simulink model "asm_blocks_lib"  (R2026b)
settings: Solver=VariableStepAuto
libraries: nesl_utility x45, asmlib_lib x25, fl_lib x3, ee_lib x3
(part 2 of 3)

== system asm_blocks_lib/Messgeräte ==
  Amperemeter : Subsystem  Tag=asmlib:ammeter  mask(ASM-Bibliothek: Amperemeter){f_meas=50}
      mask prompts: f_meas "Grundfrequenz für Effektivwerte f_mess [Hz]"
      mask help:
      | Strommesser, in Reihe schalten. Positiver Strom fließt von p nach n.
      |
      | Gleichungen:
      |   I_eff = √( f_mess·∫ i² dt )  über eine Periode 1/f_mess
      |
      | Quelle: Hagl, R.: Elektrische Antriebstechnik. Hanser, München 2013
      mask Help:
      | Strommesser, in Reihe schalten. Positiver Strom fließt von p nach n.
      | 
      | Gleichungen:
      |   I_eff = √( f_mess·∫ i² dt )  über eine Periode 1/f_mess
      | 
      | Quelle: Hagl, R.: Elektrische Antriebstechnik. Hanser, München 2013
      | 
      | Parameter und Wertebereiche:
      |   f_meas         > 0, ≤ 1000  [Hz]
      | 
      | Alle Standardwerte sind Beispielwerte (parameter/asm_standard.m), keine Datenblattwerte.
      | Spezifikation: doku/SPEC.md
      mask Display:
      | plot(0.5+0.3*cos(0:0.05:6.3), 0.5+0.3*sin(0:0.05:6.3));
      | plot([0.5 0.68], [0.5 0.68]);
      | text(0.5, 0.5, 'A', 'horizontalAlignment', 'center', 'verticalAlignment', 'middle', 'texmode', 'on');
      | port_label('LConn', 1, 'p', 'texmode', 'on');
      | port_label('RConn', 1, 'n', 'texmode', 'on');
      | port_label('output', 1, 'i', 'texmode', 'on');
      | port_label('output', 2, 'I_{eff}', 'texmode', 'on');
  Drehmomentmesswelle : Subsystem  Tag=asmlib:torque_sensor  mask(ASM-Bibliothek: Drehmomentmesswelle){}
      mask help:
      | Drehmomentmesswelle, in Reihe in den Wellenstrang schalten.
      |
      | Gleichungen:
      |   M = übertragenes Wellenmoment von R nach C
      |
      | Quelle: Hagl, R.: Elektrische Antriebstechnik. Hanser, München 2013
      mask Help:
      | Drehmomentmesswelle, in Reihe in den Wellenstrang schalten.
      | 
      | Gleichungen:
      |   M = übertragenes Wellenmoment von R nach C
      | 
      | Quelle: Hagl, R.: Elektrische Antriebstechnik. Hanser, München 2013
      | 
      | Parameter und Wertebereiche:
      |   (keine)
      | 
      | Alle Standardwerte sind Beispielwerte (parameter/asm_standard.m), keine Datenblattwerte.
      | Spezifikation: doku/SPEC.md
      mask Display:
      | plot(0.5+0.3*cos(0:0.05:6.3), 0.5+0.3*sin(0:0.05:6.3));
      | plot([0.5 0.68], [0.5 0.68]);
      | text(0.5, 0.5, 'M', 'horizontalAlignment', 'center', 'verticalAlignment', 'middle', 'texmode', 'on');
      | port_label('LConn', 1, 'R', 'texmode', 'on');
      | port_label('RConn', 1, 'C', 'texmode', 'on');
      | port_label('output', 1, 'M', 'texmode', 'on');
  Drehzahlmesser : Subsystem  Tag=asmlib:speed_sensor  mask(ASM-Bibliothek: Drehzahlmesser){ns=1500}
      mask prompts: ns "Synchrondrehzahl ns (für den Schlupf) [1/min]"
      mask help:
      | Drehzahlmesser (Tacho), parallel zwischen Welle R und Bezug C.
      |
      | Gleichungen:
      |   n = 60·Ω/(2π),  s = (ns − n)/ns
      |
      | Quelle: Hagl, R.: Elektrische Antriebstechnik. Hanser, München 2013; Densborn, Skript "DS-Asynchron-Motor" (DHBW Mannheim), Folien 45-46
      mask Help:
      | Drehzahlmesser (Tacho), parallel zwischen Welle R und Bezug C.
      | 
      | Gleichungen:
      |   n = 60·Ω/(2π),  s = (ns − n)/ns
      | 
      | Quelle: Hagl, R.: Elektrische Antriebstechnik. Hanser, München 2013; Densborn, Skript "DS-Asynchron-Motor" (DHBW Mannheim), Folien 45-46
      | 
      | Parameter und Wertebereiche:
      |   ns             > 0  [1/min]
      | 
      | Alle Standardwerte sind Beispielwerte (parameter/asm_standard.m), keine Datenblattwerte.
      | Spezifikation: doku/SPEC.md
      mask Display:
      | plot(0.5+0.3*cos(0:0.05:6.3), 0.5+0.3*sin(0:0.05:6.3));
      | plot([0.5 0.68], [0.5 0.68]);
      | text(0.5, 0.5, 'n', 'horizontalAlignment', 'center', 'verticalAlignment', 'middle', 'texmode', 'on');
      | port_label('LConn', 1, 'R', 'texmode', 'on');
      | port_label('RConn', 1, 'C', 'texmode', 'on');
      | port_label('output', 1, 'n', 'texmode', 'on');
      | port_label('output', 2, 'Om', 'texmode', 'on');
      | port_label('output', 3, '\vartheta', 'texmode', 'on');
      | port_label('output', 4, 's', 'texmode', 'on');
  Leistungsmesser 3~ : Subsystem  Tag=asmlib:power_meter3  mask(ASM-Bibliothek: Leistungsmesser 3~){f_meas=50}
      mask prompts: f_meas "Grundfrequenz für Effektivwerte f_mess [Hz]"
      mask help:
      | Dreiphasiger Leistungsmesser: Strompfade in Reihe, Spannungspfade intern gegen künstlichen Sternpunkt.
      |
      | Gleichungen:
      |   p = Σ u_k·i_k,  q = [(u_b − u_c)·i_a + (u_c − u_a)·i_b + (u_a − u_b)·i_c]/√3
      |   P, Q = Mittelwerte über 1/f_mess (Q > 0 induktiv),  S = √(ΣU_k²)·√(ΣI_k²),  cos φ = P/S
      |   symmetrisch: P = √3·U·I·cos φ,  Q = √3·U·I·sin φ,  S = √3·U·I
      |
      | Quelle: Hagl, R.: Elektrische Antriebstechnik. Hanser, München 2013; Densborn, Skript "Drehstrom & Drehfeld" (DHBW Mannheim), Folie 22
      mask Help:
      | Dreiphasiger Leistungsmesser: Strompfade in Reihe, Spannungspfade intern gegen künstlichen Sternpunkt.
      | 
      | Gleichungen:
      |   p = Σ u_k·i_k,  q = [(u_b − u_c)·i_a + (u_c − u_a)·i_b + (u_a − u_b)·i_c]/√3
      |   P, Q = Mittelwerte über 1/f_mess (Q > 0 induktiv),  S = √(ΣU_k²)·√(ΣI_k²),  cos φ = P/S
      |   symmetrisch: P = √3·U·I·cos φ,  Q = √3·U·I·sin φ,  S = √3·U·I
      | 
      | Quelle: Hagl, R.: Elektrische Antriebstechnik. Hanser, München 2013; Densborn, Skript "Drehstrom & Drehfeld" (DHBW Mannheim), Folie 22
      | 
      | Parameter und Wertebereiche:
      |   f_meas         > 0, ≤ 1000  [Hz]
      | 
      | Alle Standardwerte sind Beispielwerte (parameter/asm_standard.m), keine Datenblattwerte.
      | Spezifikation: doku/SPEC.md
      mask Display:
      | plot(0.5+0.3*cos(0:0.05:6.3), 0.5+0.3*sin(0:0.05:6.3));
      | plot([0.5 0.68], [0.5 0.68]);
      | text(0.5, 0.5, 'W', 'horizontalAlignment', 'center', 'verticalAlignment', 'middle', 'texmode', 'on');
      | port_label('LConn', 1, 'a\_in', 'texmode', 'on');
      | port_label('LConn', 2, 'b\_in', 'texmode', 'on');
      | port_label('LConn', 3, 'c\_in', 'texmode', 'on');
      | port_label('RConn', 1, 'a\_out', 'texmode', 'on');
      | port_label('RConn', 2, 'b\_out', 'texmode', 'on');
      | port_label('RConn', 3, 'c\_out', 'texmode', 'on');
      | port_label('output', 1, 'P', 'texmode', 'on');
      | port_label('output', 2, 'Q', 'texmode', 'on');
      | port_label('output', 3, 'S', 'texmode', 'on');
      | port_label('output', 4, 'cosphi', 'texmode', 'on');
  Luftspalt-Sonde : Subsystem  Tag=asmlib:airgap_probe  mask(ASM-Bibliothek: Luftspalt-Sonde){p=2, N1xi1=144, l=0.15, r=0.06}
      mask prompts: p "Polpaarzahl p [-]"; N1xi1 "wirksame Windungszahl N1·ξ1 [-]"; l "wirksame Stablänge l [m]"; r "Radius der Stabmitte r [m]"
      mask help:
      | Misst das Drehfeld im Luftspalt (wie eine Hallsonde), parallel am Port LS anschließen.
      |
      | Gleichungen:
      |   ψh = Across-Größe am Port LS
      |   φ_el = ∠ψh,   B̂ = p·|ψh| / (2·N1ξ1·l·r),   B(γ,t) = B̂·cos(γ − φ_el)
      |
      | Quelle: Hagl, R.: Elektrische Antriebstechnik. Hanser, München 2013; Densborn, Skript "DS-Asynchron-Motor" (DHBW Mannheim), Folie 14
      mask Help:
      | Misst das Drehfeld im Luftspalt (wie eine Hallsonde), parallel am Port LS anschließen.
      | 
      | Gleichungen:
      |   ψh = Across-Größe am Port LS
      |   φ_el = ∠ψh,   B̂ = p·|ψh| / (2·N1ξ1·l·r),   B(γ,t) = B̂·cos(γ − φ_el)
      | 
      | Quelle: Hagl, R.: Elektrische Antriebstechnik. Hanser, München 2013; Densborn, Skript "DS-Asynchron-Motor" (DHBW Mannheim), Folie 14
      | 
      | Parameter und Wertebereiche:
      |   p              ganzzahlig, ≥ 1, ≤ 12  [-]
      |   N1xi1          > 0  [-]
      |   l              > 0  [m]
      |   r              > 0  [m]
      | 
      | Alle Standardwerte sind Beispielwerte (parameter/asm_standard.m), keine Datenblattwerte.
      | Spezifikation: doku/SPEC.md
      mask Display:
      | plot(0.5+0.3*cos(0:0.05:6.3), 0.5+0.3*sin(0:0.05:6.3));
      | plot([0.5 0.68], [0.5 0.68]);
      | text(0.5, 0.5, 'B', 'horizontalAlignment', 'center', 'verticalAlignment', 'middle', 'texmode', 'on');
      | port_label('LConn', 1, 'LS', 'texmode', 'on');
      | port_label('output', 1, '\psi_h', 'texmode', 'on');
      | port_label('output', 2, '\phi_{el}', 'texmode', 'on');
      | port_label('output', 3, 'Bhat', 'texmode', 'on');
  Schreiber : Subsystem  Tag=asmlib:recorder  mask(ASM-Bibliothek: Schreiber){title_text=Messung}
      mask prompts: title_text "Titel (erscheint auf dem Baustein)"
      mask help:
      | Messschreiber (Simulink Scope). Mehrere Signale über einen Mux anschließen; das Scope zeigt
      | die Signalnamen. Für Folienbilder die Signale protokollieren und mit asmexport.slide_figure exportieren.
      |
      | Gleichungen:
      |   –
      |
      | Quelle: Hagl, R.: Elektrische Antriebstechnik. Hanser, München 2013
      mask Help:
      | Messschreiber (Simulink Scope). Mehrere Signale über einen Mux anschließen; das Scope zeigt
      | die Signalnamen. Für Folienbilder die Signale protokollieren und mit asmexport.slide_figure exportieren.
      | 
      | Gleichungen:
      |   –
      | 
      | Quelle: Hagl, R.: Elektrische Antriebstechnik. Hanser, München 2013
      | 
      | Parameter und Wertebereiche:
      |   title_text     Text
      | 
      | Alle Standardwerte sind Beispielwerte (parameter/asm_standard.m), keine Datenblattwerte.
      | Spezifikation: doku/SPEC.md
      mask Display:
      | plot(0.5+0.3*cos(0:0.05:6.3), 0.5+0.3*sin(0:0.05:6.3));
      | plot([0.5 0.68], [0.5 0.68]);
      | text(0.5, 0.6, 'Schreiber', 'horizontalAlignment', 'center');
      | text(0.5, 0.3, title_text, 'horizontalAlignment', 'center');
      | port_label('input', 1, 'u', 'texmode', 'on');
  Spannungsmessung 3~ : Subsystem  Tag=asmlib:voltage_sensor3  mask(ASM-Bibliothek: Spannungsmessung 3~){f_meas=50, reference=künstlicher Sternpunkt}
      mask prompts: f_meas "Grundfrequenz für Effektivwerte f_mess [Hz]"; reference "Bezug der Strangspannungen"
      mask help:
      | Dreiphasige Spannungsmessung, parallel anschließen. Strangspannungen gegen den künstlichen
      | Sternpunkt oder gegen den Anschluss n (dann muss n angeschlossen sein). U_eff = Leiterspannung.
      |
      | Gleichungen:
      |   u_Str,k = v_k − v_m,  v_m = (v_a + v_b + v_c)/3 bzw. v_n;  u_ab = v_a − v_b, …
      |   U_eff = √(f_mess/3·∫(u_ab² + u_bc² + u_ca²) dt);  symmetrisch U = √3·U_Str
      |
      | Quelle: Hagl, R.: Elektrische Antriebstechnik. Hanser, München 2013; Densborn, Skript "Drehstrom & Drehfeld" (DHBW Mannheim), Folien 11-16
      mask Help:
      | Dreiphasige Spannungsmessung, parallel anschließen. Strangspannungen gegen den künstlichen
      | Sternpunkt oder gegen den Anschluss n (dann muss n angeschlossen sein). U_eff = Leiterspannung.
      | 
      | Gleichungen:
      |   u_Str,k = v_k − v_m,  v_m = (v_a + v_b + v_c)/3 bzw. v_n;  u_ab = v_a − v_b, …
      |   U_eff = √(f_mess/3·∫(u_ab² + u_bc² + u_ca²) dt);  symmetrisch U = √3·U_Str
      | 
      | Quelle: Hagl, R.: Elektrische Antriebstechnik. Hanser, München 2013; Densborn, Skript "Drehstrom & Drehfeld" (DHBW Mannheim), Folien 11-16
      | 
      | Parameter und Wertebereiche:
      |   f_meas         > 0, ≤ 1000  [Hz]
      |   reference      Auswahl: künstlicher Sternpunkt | Anschluss n
      | 
      | Alle Standardwerte sind Beispielwerte (parameter/asm_standard.m), keine Datenblattwerte.
      | Spezifikation: doku/SPEC.md
      mask TypeOptions reference: künstlicher Sternpunkt | Anschluss n
      mask Display:
      | plot(0.5+0.3*cos(0:0.05:6.3), 0.5+0.3*sin(0:0.05:6.3));
      | plot([0.5 0.68], [0.5 0.68]);
      | text(0.5, 0.5, 'V 3~', 'horizontalAlignment', 'center', 'verticalAlignment', 'middle', 'texmode', 'on');
      | port_label('LConn', 1, 'a', 'texmode', 'on');
      | port_label('LConn', 2, 'b', 'texmode', 'on');
      | port_label('LConn', 3, 'c', 'texmode', 'on');
      | port_label('LConn', 4, 'n', 'texmode', 'on');
      | port_label('output', 1, 'u_{phase}', 'texmode', 'on');
      | port_label('output', 2, 'u_{line}', 'texmode', 'on');
      | port_label('output', 3, 'U_{eff}', 'texmode', 'on');
  Strommessung 3~ : Subsystem  Tag=asmlib:current_sensor3  mask(ASM-Bibliothek: Strommessung 3~){f_meas=50}
      mask prompts: f_meas "Grundfrequenz für Effektivwerte f_mess [Hz]"
      mask help:
      | Dreiphasige Strommessung, in Reihe in die drei Leiter schalten.
      |
      | Gleichungen:
      |   i1 = 2/3·(i_a + a·i_b + a²·i_c)  (Raumzeiger)
      |   I_eff = √(f_mess/3·∫(i_a² + i_b² + i_c²) dt)  (quadratischer Mittelwert der drei Leiter)
      |
      | Quelle: Hagl, R.: Elektrische Antriebstechnik. Hanser, München 2013; Densborn, Skript "Drehstrom & Drehfeld" (DHBW Mannheim)
      mask Help:
      | Dreiphasige Strommessung, in Reihe in die drei Leiter schalten.
      | 
      | Gleichungen:
      |   i1 = 2/3·(i_a + a·i_b + a²·i_c)  (Raumzeiger)
      |   I_eff = √(f_mess/3·∫(i_a² + i_b² + i_c²) dt)  (quadratischer Mittelwert der drei Leiter)
      | 
      | Quelle: Hagl, R.: Elektrische Antriebstechnik. Hanser, München 2013; Densborn, Skript "Drehstrom & Drehfeld" (DHBW Mannheim)
      | 
      | Parameter und Wertebereiche:
      |   f_meas         > 0, ≤ 1000  [Hz]
      | 
      | Alle Standardwerte sind Beispielwerte (parameter/asm_standard.m), keine Datenblattwerte.
      | Spezifikation: doku/SPEC.md
      mask Display:
      | plot(0.5+0.3*cos(0:0.05:6.3), 0.5+0.3*sin(0:0.05:6.3));
      | plot([0.5 0.68], [0.5 0.68]);
      | text(0.5, 0.5, 'A 3~', 'horizontalAlignment', 'center', 'verticalAlignment', 'middle', 'texmode', 'on');
      | port_label('LConn', 1, 'a\_in', 'texmode', 'on');
      | port_label('LConn', 2, 'b\_in', 'texmode', 'on');
      | port_label('LConn', 3, 'c\_in', 'texmode', 'on');
      | port_label('RConn', 1, 'a\_out', 'texmode', 'on');
      | port_label('RConn', 2, 'b\_out', 'texmode', 'on');
      | port_label('RConn', 3, 'c\_out', 'texmode', 'on');
      | port_label('output', 1, 'i_{abc}', 'texmode', 'on');
      | port_label('output', 2, 'I_{eff}', 'texmode', 'on');
      | port_label('output', 3, 'i1', 'texmode', 'on');
  Voltmeter : Subsystem  Tag=asmlib:voltmeter  mask(ASM-Bibliothek: Voltmeter){f_meas=50}
      mask prompts: f_meas "Grundfrequenz für Effektivwerte f_mess [Hz]"
      mask help:
      | Spannungsmesser, parallel schalten. u = v_p − v_n.
      |
      | Gleichungen:
      |   U_eff = √( f_mess·∫ u² dt )  über eine Periode 1/f_mess
      |
      | Quelle: Hagl, R.: Elektrische Antriebstechnik. Hanser, München 2013
      mask Help:
      | Spannungsmesser, parallel schalten. u = v_p − v_n.
      | 
      | Gleichungen:
      |   U_eff = √( f_mess·∫ u² dt )  über eine Periode 1/f_mess
      | 
      | Quelle: Hagl, R.: Elektrische Antriebstechnik. Hanser, München 2013
      | 
      | Parameter und Wertebereiche:
      |   f_meas         > 0, ≤ 1000  [Hz]
      | 
      | Alle Standardwerte sind Beispielwerte (parameter/asm_standard.m), keine Datenblattwerte.
      | Spezifikation: doku/SPEC.md
      mask Display:
      | plot(0.5+0.3*cos(0:0.05:6.3), 0.5+0.3*sin(0:0.05:6.3));
      | plot([0.5 0.68], [0.5 0.68]);
      | text(0.5, 0.5, 'V', 'horizontalAlignment', 'center', 'verticalAlignment', 'middle', 'texmode', 'on');
      | port_label('LConn', 1, 'p', 'texmode', 'on');
      | port_label('RConn', 1, 'n', 'texmode', 'on');
      | port_label('output', 1, 'u', 'texmode', 'on');
      | port_label('output', 2, 'U_{eff}', 'texmode', 'on');

== system asm_blocks_lib/Quellen ==
  Netz 3~ : Subsystem  Tag=asmlib:grid3  mask(ASM-Bibliothek: Netz 3~){U_L=400, f1=50, phase_seq=L1-L2-L3 (Rechtsdrehfeld), phi0=0, t_on=0, R_N=0, L_N=0}
      mask prompts: U_L "Leiterspannung U (Effektivwert) [V]"; f1 "Frequenz f1 [Hz]"; phase_seq "Phasenfolge"; phi0 "Nullphasenwinkel von L1 [°]"; t_on "Einschaltzeitpunkt t_ein [s]"; R_N "Netzinnenwiderstand je Leiter R_N [Ω]"; L_N "Netzinneninduktivität je Leiter L_N [H]"
      mask help:
      | Symmetrisches Drehstromnetz, Sternpunkt n herausgeführt, optional mit Innenimpedanz (R_N = L_N = 0: starres Netz).
      |
      | Gleichungen:
      |   u_L1 = √2·U/√3·sin(ω1·t + φ0),  u_L2 = √2·U/√3·sin(ω1·t + φ0 − 2π/3),
      |   u_L3 = √2·U/√3·sin(ω1·t + φ0 − 4π/3)  (Rechtsdrehfeld),  ω1 = 2π·f1
      |   Spannung liegt ab t ≥ t_ein an.
      |
      | Quelle: Hagl, R.: Elektrische Antriebstechnik. Hanser, München 2013; Densborn, Skript "Drehstrom & Drehfeld" (DHBW Mannheim), Folien 8-12
      mask Help:
      | Symmetrisches Drehstromnetz, Sternpunkt n herausgeführt, optional mit Innenimpedanz (R_N = L_N = 0: starres Netz).
      | 
      | Gleichungen:
      |   u_L1 = √2·U/√3·sin(ω1·t + φ0),  u_L2 = √2·U/√3·sin(ω1·t + φ0 − 2π/3),
      |   u_L3 = √2·U/√3·sin(ω1·t + φ0 − 4π/3)  (Rechtsdrehfeld),  ω1 = 2π·f1
      |   Spannung liegt ab t ≥ t_ein an.
      | 
      | Quelle: Hagl, R.: Elektrische Antriebstechnik. Hanser, München 2013; Densborn, Skript "Drehstrom & Drehfeld" (DHBW Mannheim), Folien 8-12
      | 
      | Parameter und Wertebereiche:
      |   U_L            ≥ 0, ≤ 1e4  [V]
      |   f1             > 0, ≤ 1000  [Hz]
      |   phase_seq      Auswahl: L1-L2-L3 (Rechtsdrehfeld) | L1-L3-L2 (Linksdrehfeld)
      |   phi0           ≥ -360, ≤ 360  [°]
      |   t_on           ≥ 0  [s]
      |   R_N            ≥ 0  [Ω]
      |   L_N            ≥ 0  [H]
      | 
      | Alle Standardwerte sind Beispielwerte (parameter/asm_standard.m), keine Datenblattwerte.
      | Spezifikation: doku/SPEC.md
      mask TypeOptions phase_seq: L1-L2-L3 (Rechtsdrehfeld) | L1-L3-L2 (Linksdrehfeld)
      mask Display:
      | plot(0.5+0.3*cos(0:0.05:6.3), 0.5+0.3*sin(0:0.05:6.3));
      | text(0.5, 0.5, '3~', 'horizontalAlignment', 'center', 'verticalAlignment', 'middle', 'texmode', 'on');
      | port_label('RConn', 1, 'a', 'texmode', 'on');
      | port_label('RConn', 2, 'b', 'texmode', 'on');
      | port_label('RConn', 3, 'c', 'texmode', 'on');
      | port_label('RConn', 4, 'n', 'texmode', 'on');
  Sternpunkt (Erde) : Subsystem  Tag=asmlib:neutral_ground  mask(ASM-Bibliothek: Sternpunkt (Erde)){}
      mask help:
      | Elektrisches Bezugspotenzial (0 V). Jedes elektrische Netzwerk braucht mindestens einen Bezug.
      |
      | Gleichungen:
      |   u_N = 0
      |
      | Quelle: Hagl, R.: Elektrische Antriebstechnik. Hanser, München 2013
      mask Help:
      | Elektrisches Bezugspotenzial (0 V). Jedes elektrische Netzwerk braucht mindestens einen Bezug.
      | 
      | Gleichungen:
      |   u_N = 0
      | 
      | Quelle: Hagl, R.: Elektrische Antriebstechnik. Hanser, München 2013
      | 
      | Parameter und Wertebereiche:
      |   (keine)
      | 
      | Alle Standardwerte sind Beispielwerte (parameter/asm_standard.m), keine Datenblattwerte.
      | Spezifikation: doku/SPEC.md
      mask Display:
      | plot(0.5+0.3*cos(0:0.05:6.3), 0.5+0.3*sin(0:0.05:6.3));
      | text(0.5, 0.5, '\perp', 'horizontalAlignment', 'center', 'verticalAlignment', 'middle', 'texmode', 'on');
      | port_label('LConn', 1, 'N', 'texmode', 'on');

== system asm_blocks_lib/Referenz ==
  ASM Kloss (quasistationär) : Subsystem  Tag=asmlib:asm_kloss  mask(ASM-Bibliothek: ASM Kloss (quasistationär)){MK=71.55, sK=0.2, ns=1500}
      mask prompts: MK "Kippmoment MK [N·m]"; sK "Kippschlupf sK [-]"; ns "Synchrondrehzahl ns [1/min]"
      mask help:
      | Quasistationäres Motormoment nach Kloss (Teil B des Prototyps, R1 = 0, konstanter Fluss,
      | keine elektrische Dynamik, keine eigene Trägheit: J_M als Schwungmasse anschließen).
      |
      | Gleichungen:
      |   M = 2·MK·s·sK / (s² + sK²),   s = (ns − n)/ns
      |
      | Quelle: Hagl, R.: Elektrische Antriebstechnik. Hanser, München 2013; Densborn, Skript "DS-Asynchron-Motor" (DHBW Mannheim), Folien 47-50
      mask Help:
      | Quasistationäres Motormoment nach Kloss (Teil B des Prototyps, R1 = 0, konstanter Fluss,
      | keine elektrische Dynamik, keine eigene Trägheit: J_M als Schwungmasse anschließen).
      | 
      | Gleichungen:
      |   M = 2·MK·s·sK / (s² + sK²),   s = (ns − n)/ns
      | 
      | Quelle: Hagl, R.: Elektrische Antriebstechnik. Hanser, München 2013; Densborn, Skript "DS-Asynchron-Motor" (DHBW Mannheim), Folien 47-50
      | 
      | Parameter und Wertebereiche:
      |   MK             > 0  [N·m]
      |   sK             > 0, ≤ 1  [-]
      |   ns             > 0  [1/min]
      | 
      | Alle Standardwerte sind Beispielwerte (parameter/asm_standard.m), keine Datenblattwerte.
      | Spezifikation: doku/SPEC.md
      mask Display:
      | plot([0.1 0.9], [0.1 0.1]); plot([0.1 0.9], [0.9 0.9]);
      | text(0.5, 0.5, 'Kloss', 'horizontalAlignment', 'center', 'verticalAlignment', 'middle', 'texmode', 'on');
      | port_label('RConn', 1, 'R', 'texmode', 'on');
      | port_label('RConn', 2, 'C', 'texmode', 'on');
      | port_label('output', 1, 'M', 'texmode', 'on');
      | port_label('output', 2, 's', 'texmode', 'on');
  ASM Referenz (Simscape Electrical) : Subsystem  Tag=asmlib:asm_reference  mask(ASM-Bibliothek: ASM Referenz (Simscape Electrical)){param_set=Standard, U_N=400, f_N=50, p=2, R1=0.5, L1s=0.009902, Lh=0.25, R2b=1.225, L2sb=0.009902, J_M=0.012}
      mask prompts: param_set "Parametersatz"; U_N "Bemessungsspannung U_N (Leiter, eff.) [V]"; f_N "Bemessungsfrequenz f_N [Hz]"; p "Polpaarzahl p [-]"; R1 "Statorwiderstand R1 [Ω]"; L1s "Statorstreuinduktivität L1σ [H]"; Lh "Hauptinduktivität Lh [H]"; R2b "Rotorwiderstand R2′ (statorbezogen) [Ω]"; L2sb "Rotorstreuinduktivität L2σ′ (statorbezogen) [H]"; J_M "Trägheitsmoment Motor J_M [kg·m²]"
      mask help:
      | Referenzmotor mit "Induction Machine Squirrel Cage" aus Simscape Electrical (ee_lib) und demselben
      | Parametersatz wie "ASM Standard" (Sternschaltung, Sternpunkt frei, Start stromlos). J_M liegt als
      | Schwungmasse an der Welle R. Nur zum Modellvergleich (Benchmark), keine Messung.
      | Hinweis: Die ee_lib-Maschine verträgt keine Solver-Ereignisse (Sprünge, unstetige Funktionen)
      | im selben Modell; alle Bausteine der Bibliothek sind deshalb ereignisfrei formuliert.
      |
      | Gleichungen:
      | Raumzeigermodell, statorfest (Index 1 = Stator, 2 = Rotor, ′ = statorbezogen):
      |   u1 = R1·i1 + dψ1/dt
      |   0  = R2′·i2′ + dψ2′/dt − j·p·Ω·ψ2′
      |   ψ1 = L1σ·i1 + ψh,   ψ2′ = L2σ′·i2′ + ψh,   ψh = Lh·(i1 + i2′)
      |   M  = 3/2·p·Im{ψh*·i1},   J·dΩ/dt = M − M_L − k_R·Ω
      |   n = 60·Ω/(2π),   s = (ns − n)/ns,   ns = 60·f1/p
      |
      | Quelle: Hagl, R.: Elektrische Antriebstechnik. Hanser, München 2013
      mask init:
      | % parameter set "Standard": values from parameter/asm_standard.m
      | if param_set == 1
      |     S = asm_standard();
      |     U_N = S.U_N; f_N = S.f_N; p = S.p; R1 = S.R1; L1s = S.L1s; Lh = S.Lh; R2b = S.R2b; L2sb = S.L2sb; J_M = S.J_M;
      | end
      mask Help:
      | Referenzmotor mit "Induction Machine Squirrel Cage" aus Simscape Electrical (ee_lib) und demselben
      | Parametersatz wie "ASM Standard" (Sternschaltung, Sternpunkt frei, Start stromlos). J_M liegt als
      | Schwungmasse an der Welle R. Nur zum Modellvergleich (Benchmark), keine Messung.
      | Hinweis: Die ee_lib-Maschine verträgt keine Solver-Ereignisse (Sprünge, unstetige Funktionen)
      | im selben Modell; alle Bausteine der Bibliothek sind deshalb ereignisfrei formuliert.
      | 
      | Gleichungen:
      | Raumzeigermodell, statorfest (Index 1 = Stator, 2 = Rotor, ′ = statorbezogen):
      |   u1 = R1·i1 + dψ1/dt
      |   0  = R2′·i2′ + dψ2′/dt − j·p·Ω·ψ2′
      |   ψ1 = L1σ·i1 + ψh,   ψ2′ = L2σ′·i2′ + ψh,   ψh = Lh·(i1 + i2′)
      |   M  = 3/2·p·Im{ψh*·i1},   J·dΩ/dt = M − M_L − k_R·Ω
      |   n = 60·Ω/(2π),   s = (ns − n)/ns,   ns = 60·f1/p
      | 
      | Quelle: Hagl, R.: Elektrische Antriebstechnik. Hanser, München 2013
      | 
      | Parameter und Wertebereiche:
      |   param_set      Auswahl: Standard | Benutzerdefiniert
      |   U_N            > 0, ≤ 1e4  [V]
      |   f_N            > 0, ≤ 1000  [Hz]
      |   p              ganzzahlig, ≥ 1, ≤ 12  [-]
      |   R1             > 0  [Ω]
      |   L1s            > 0  [H]
      |   Lh             > 0  [H]
      |   R2b            > 0  [Ω]
      |   L2sb           > 0  [H]
      |   J_M            > 0  [kg·m²]
      | 
      | Alle Standardwerte sind Beispielwerte (parameter/asm_standard.m), keine Datenblattwerte.
      | Spezifikation: doku/SPEC.md
      mask TypeOptions param_set: Standard | Benutzerdefiniert
      mask Callback param_set: asmtools.param_set_callback(gcb);
      mask Display:
      | plot([0.1 0.9], [0.1 0.1]); plot([0.1 0.9], [0.9 0.9]);
      | text(0.5, 0.5, 'Referenz', 'horizontalAlignment', 'center', 'verticalAlignment', 'middle', 'texmode', 'on');
      | port_label('LConn', 1, 'a', 'texmode', 'on');
      | port_label('LConn', 2, 'b', 'texmode', 'on');
      | port_label('LConn', 3, 'c', 'texmode', 'on');
      | port_label('RConn', 1, 'R', 'texmode', 'on');
      | port_label('RConn', 2, 'C', 'texmode', 'on');
  Leiterschleife (Prototyp Teil A) : Subsystem  Tag=asmlib:conductor_loop  mask(ASM-Bibliothek: Leiterschleife (Prototyp Teil A)){Bhat=0.8, l=0.15, r=0.06, f1=50, p=2, R2_S=0.000318664, L2s_S=5.0717e-06, conv_phi2=+1, phi2_mode=aus Rotorimpedanz, phi2_fix=90}
      mask prompts: Bhat "Amplitude der Luftspaltflussdichte B̂ [T]"; l "wirksame Stablänge l [m]"; r "Radius der Stabmitte r [m]"; f1 "Statorfrequenz f1 [Hz]"; p "Polpaarzahl p [-]"; R2_S "Widerstand der Leiterschleife R2 [Ω]"; L2s_S "Streuinduktivität der Leiterschleife L2σ [H]"; conv_phi2 "Vorzeichenkonvention konv_phi2"; phi2_mode "Versatzwinkel φ2"; phi2_fix "fester Versatzwinkel φ2 [°]"
      mask help:
      | Leiterschleife aus zwei Rotorstäben im rotorfesten System (Teil A des Prototyps), Eingang Schlupf s.
      | Der Schlupf ist eine Vorgabe (Konstante oder Signal); das Schleifenmoment wirkt nicht auf die Mechanik
      | zurück. R2 und L2σ sind aus MK und sK abgeleitet (parameter/asm_standard.m).
      |
      | Gleichungen:
      |   θ2 = ∫ s·ω1 dt,  B_k = B̂·cos(γ_k − θ2),  i_k = î2·sin(γ_k − θ2 + konv·φ2)
      |   F_k = konv·i_k·l·B_k,  M_k = F_k·r,  M_S = M_1 + M_2
      |
      | Quelle: Hagl, R.: Elektrische Antriebstechnik. Hanser, München 2013; Densborn, Skript "DS-Asynchron-Motor" (DHBW Mannheim), Folien 14-16
      mask Help:
      | Leiterschleife aus zwei Rotorstäben im rotorfesten System (Teil A des Prototyps), Eingang Schlupf s.
      | Der Schlupf ist eine Vorgabe (Konstante oder Signal); das Schleifenmoment wirkt nicht auf die Mechanik
      | zurück. R2 und L2σ sind aus MK und sK abgeleitet (parameter/asm_standard.m).
      | 
      | Gleichungen:
      |   θ2 = ∫ s·ω1 dt,  B_k = B̂·cos(γ_k − θ2),  i_k = î2·sin(γ_k − θ2 + konv·φ2)
      |   F_k = konv·i_k·l·B_k,  M_k = F_k·r,  M_S = M_1 + M_2
      | 
      | Quelle: Hagl, R.: Elektrische Antriebstechnik. Hanser, München 2013; Densborn, Skript "DS-Asynchron-Motor" (DHBW Mannheim), Folien 14-16
      | 
      | Parameter und Wertebereiche:
      |   Bhat           > 0, ≤ 2.5  [T]
      |   l              > 0  [m]
      |   r              > 0  [m]
      |   f1             > 0, ≤ 1000  [Hz]
      |   p              ganzzahlig, ≥ 1, ≤ 12  [-]
      |   R2_S           > 0  [Ω]
      |   L2s_S          > 0  [H]
      |   conv_phi2      Auswahl: +1 | -1
      |   phi2_mode      Auswahl: aus Rotorimpedanz | fest
      |   phi2_fix       ≥ 0, ≤ 180  [°]
      | 
      | Alle Standardwerte sind Beispielwerte (parameter/asm_standard.m), keine Datenblattwerte.
      | Spezifikation: doku/SPEC.md
      mask TypeOptions conv_phi2: +1 | -1
      mask TypeOptions phi2_mode: aus Rotorimpedanz | fest
      mask Display:
      | plot([0.1 0.9], [0.1 0.1]); plot([0.1 0.9], [0.9 0.9]);
      | text(0.5, 0.5, 'Schleife', 'horizontalAlignment', 'center', 'verticalAlignment', 'middle', 'texmode', 'on');
      | port_label('input', 1, 's', 'texmode', 'on');
      | port_label('output', 1, 'B_k', 'texmode', 'on');
      | port_label('output', 2, 'i_k', 'texmode', 'on');
      | port_label('output', 3, 'F_k', 'texmode', 'on');
      | port_label('output', 4, 'M_k', 'texmode', 'on');
      | port_label('output', 5, 'M_S', 'texmode', 'on');
      | port_label('output', 6, 'B_\perp', 'texmode', 'on');
      | port_label('output', 7, '\phi2', 'texmode', 'on');
      | port_label('output', 8, 'i2hat', 'texmode', 'on');
      | port_label('output', 9, '\theta_2', 'texmode', 'on');

== system asm_blocks_lib/Didaktik/Drehfeld-Anzeige ==
  psi_h : Inport
  i2b : Inport  Port=2
  th_mech : Inport  Port=3
  Log : ToWorkspace  VariableName=field_display_log  SaveFormat=Structure With Time  SampleTime=-1
  Mux : Mux  Inputs=[2 2 1]
  wires:
  psi_h/1 -> Mux/1
  i2b/1 -> Mux/2
  th_mech/1 -> Mux/3
  Mux/1 -> Log/1

== system asm_blocks_lib/Didaktik/Ideales Drehfeld ==
  Clock : Clock
  Field : MATLABSystem  System=asmtools.IdealRotatingField  Bhat=Bhat  f1=f1  p=p  s=s  l=l  r=r  N1xi1=N1xi1  N2=N2  R2_S=R2_S  L2s_S=L2s_S  mode=phi2_mode  phi2_fix=phi2_fix  SimulateUsing=Interpreted execution
      mask Type: asmtools.IdealRotatingField
  psi_h : Outport
  i2b : Outport  Port=2
  th_mech : Outport  Port=3
  phi_el : Outport  Port=4
  phi2 : Outport  Port=5
  wires:
  Clock/1 -> Field/1
  Field/1 -> psi_h/1
  Field/2 -> i2b/1
  Field/3 -> th_mech/1
  Field/4 -> phi_el/1
  Field/5 -> phi2/1

== system asm_blocks_lib/Didaktik/Kennlinienschreiber ==
  n : Inport
  M : Inport  Port=2
  M_L : Inport  Port=3
  Log : ToWorkspace  VariableName=torque_speed_log  SaveFormat=Structure With Time  SampleTime=-1
  Mux : Mux  Inputs=3
  wires:
  n/1 -> Mux/1
  M/1 -> Mux/2
  M_L/1 -> Mux/3
  Mux/1 -> Log/1

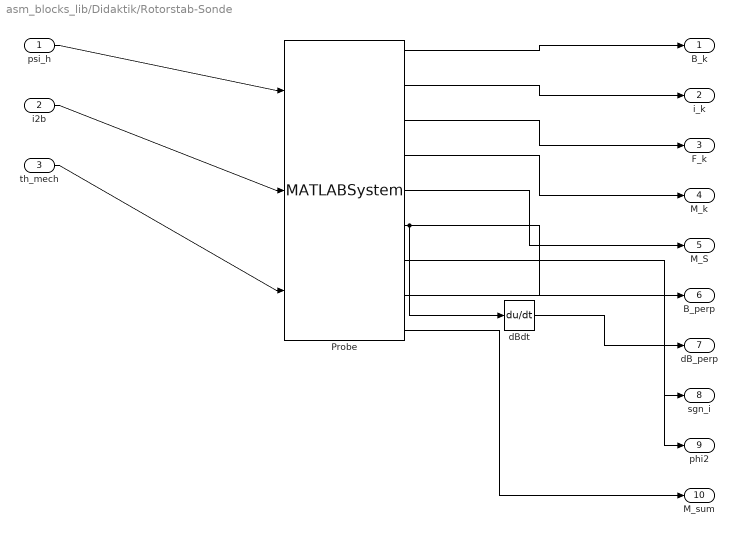
== system asm_blocks_lib/Didaktik/Rotorstab-Sonde ==
  psi_h : Inport
  i2b : Inport  Port=2
  th_mech : Inport  Port=3
  Probe : MATLABSystem  System=asmtools.RotorBarProbe  p=p  N2=N2  l=l  r=r  N1xi1=N1xi1  k1=k1  k2=k2  bar1_angle=bar1_angle*pi/180  slide_convention=convention == 1  SimulateUsing=Interpreted execution
      mask Type: asmtools.RotorBarProbe
  dBdt : Derivative
  B_k : Outport
  i_k : Outport  Port=2
  F_k : Outport  Port=3
  M_k : Outport  Port=4
  M_S : Outport  Port=5
  B_perp : Outport  Port=6
  dB_perp : Outport  Port=7
  sgn_i : Outport  Port=8
  phi2 : Outport  Port=9
  M_sum : Outport  Port=10
  wires:
  psi_h/1 -> Probe/1
  i2b/1 -> Probe/2
  th_mech/1 -> Probe/3
  Probe/6 -> dBdt/1, B_perp/1
  Probe/1 -> B_k/1
  Probe/2 -> i_k/1
  Probe/3 -> F_k/1
  Probe/4 -> M_k/1
  Probe/5 -> M_S/1
  dBdt/1 -> dB_perp/1
  Probe/7 -> sgn_i/1
  Probe/8 -> phi2/1
  Probe/9 -> M_sum/1

== system asm_blocks_lib/Didaktik/Spulenfelder ==
  i_abc : Inport
  f_BUVW : Gain  Gain=p*Lh/(2*N1xi1*l*r)*2/3
  f_Bhat : Fcn  Expr=p*Lh/(2*N1xi1*l*r)*sqrt((2/3*(u(1)-u(2)/2-u(3)/2))^2 + ((u(2)-u(3))/sqrt(3))^2)
  f_phi : Fcn  Expr=atan2((u(2)-u(3))/sqrt(3), 2/3*(u(1)-u(2)/2-u(3)/2))
  B_UVW : Outport
  Bhat : Outport  Port=2
  phi_el : Outport  Port=3
  wires:
  i_abc/1 -> f_BUVW/1, f_Bhat/1, f_phi/1
  f_BUVW/1 -> B_UVW/1
  f_Bhat/1 -> Bhat/1
  f_phi/1 -> phi_el/1

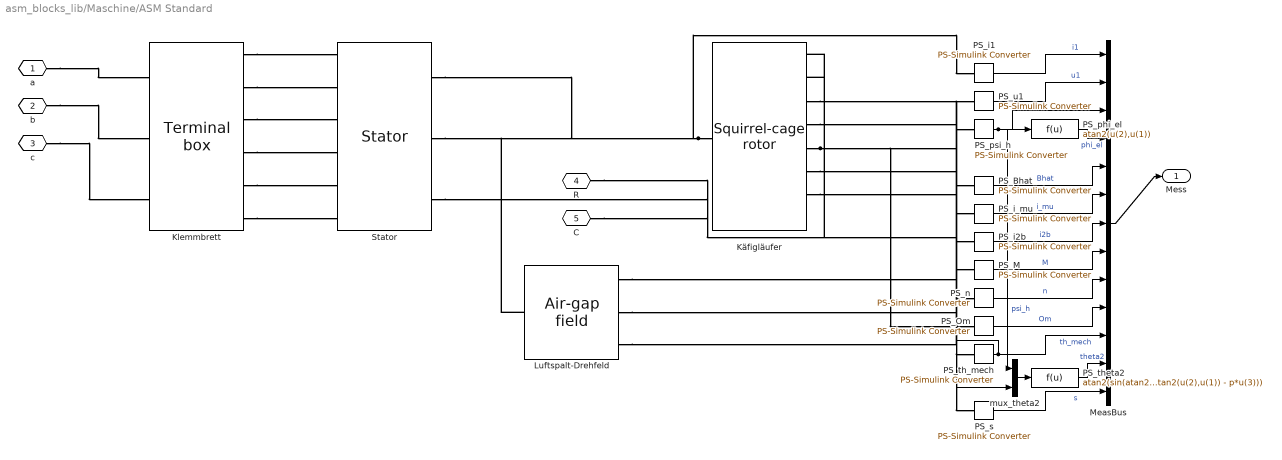
== system asm_blocks_lib/Maschine/ASM Standard ==
  Klemmbrett : asmlib_lib/machine/Terminal box  connection=connection  i_aU1_specify=off  i_aU1_priority=None  i_aU1=0 A  i_aU1_nominal_specify=off  i_aU1_nominal_value=1  i_aU1_nominal_unit=A  i_bV1_specify=off  i_bV1_priority=None  i_bV1=0 A  i_bV1_nominal_specify=off  i_bV1_nominal_value=1  i_bV1_nominal_unit=A  i_cW1_specify=off  i_cW1_priority=None  i_cW1=0 A  i_cW1_nominal_specify=off  i_cW1_nominal_value=1  i_cW1_nominal_unit=A  i_aW2_specify=off  i_aW2_priority=None  i_aW2=0 A  i_aW2_nominal_specify=off  i_aW2_nominal_value=1  i_aW2_nominal_unit=A  i_bU2_specify=off  i_bU2_priority=None  i_bU2=0 A  i_bU2_nominal_specify=off  i_bU2_nominal_value=1  i_bU2_nominal_unit=A  i_cV2_specify=off  i_cV2_priority=None  i_cV2=0 A  i_cV2_nominal_specify=off  i_cV2_nominal_value=1  i_cV2_nominal_unit=A  i_UV2_specify=off  i_UV2_priority=None  i_UV2=0 A  i_UV2_nominal_specify=off  i_UV2_nominal_value=1  i_UV2_nominal_unit=A  i_VW2_specify=off  i_VW2_priority=None  i_VW2=0 A  i_VW2_nominal_specify=off  i_VW2_nominal_value=1  i_VW2_nominal_unit=A
  Käfigläufer : asmlib_lib/machine/Squirrel-cage rotor  R2b=R2b Ohm  L2sb=L2sb H  p=p  f_N=f_N Hz  J_M=J_M kg*m^2  k_R=k_R N*m*s/rad  n0=n0 rpm  i2_specify=off  i2_priority=None  i2=zeros(2, 1) A  i2_nominal_specify=off  i2_nominal_value=1  i2_nominal_unit=A  psih_specify=off  psih_priority=None  psih=zeros(2, 1) Wb  psih_nominal_specify=off  psih_nominal_value=1  psih_nominal_unit=Wb  psi2_specify=off  psi2_priority=None  psi2=zeros(2, 1) Wb  psi2_nominal_specify=off  psi2_nominal_value=1  psi2_nominal_unit=Wb  psi2r_specify=off  psi2r_priority=High  psi2r=zeros(2, 1) Wb  psi2r_nominal_specify=off  psi2r_nominal_value=1  psi2r_nominal_unit=Wb  th_specify=off  th_priority=High  th=0 rad  th_nominal_specify=off  th_nominal_value=1  th_nominal_unit=rad  t_specify=off  t_priority=None  t=0 N*m  t_nominal_specify=off  t_nominal_value=1  t_nominal_unit=N*m  Mel_specify=off  Mel_priority=None  Mel=0 N*m  Mel_nominal_specify=off  Mel_nominal_value=1  Mel_nominal_unit=N*m
  Luftspalt-Drehfeld : asmlib_lib/machine/Air-gap field  Lh=Lh H  p=p  N1xi1=N1xi1  l=l m  r=r m  imu_specify=off  imu_priority=None  imu=zeros(2, 1) A  imu_nominal_specify=off  imu_nominal_value=1  imu_nominal_unit=A  psih_specify=off  psih_priority=None  psih=zeros(2, 1) Wb  psih_nominal_specify=off  psih_nominal_value=1  psih_nominal_unit=Wb
  MeasBus : BusCreator  Inputs=13
  PS_Bhat : nesl_utility/PS-Simulink Converter  PhysicalDomain=network_engine_domain  SubClassName=ps_output  LeftPortType=input  RightPortType=output  PseudoPeriodic=off  Frequencies=[]  VectorFormat=inherit  Unit=T  AffineConversion=off
  PS_M : nesl_utility/PS-Simulink Converter  PhysicalDomain=network_engine_domain  SubClassName=ps_output  LeftPortType=input  RightPortType=output  PseudoPeriodic=off  Frequencies=[]  VectorFormat=inherit  Unit=N*m  AffineConversion=off
  PS_Om : nesl_utility/PS-Simulink Converter  PhysicalDomain=network_engine_domain  SubClassName=ps_output  LeftPortType=input  RightPortType=output  PseudoPeriodic=off  Frequencies=[]  VectorFormat=inherit  Unit=rad/s  AffineConversion=off
  PS_i1 : nesl_utility/PS-Simulink Converter  PhysicalDomain=network_engine_domain  SubClassName=ps_output  LeftPortType=input  RightPortType=output  PseudoPeriodic=off  Frequencies=[]  VectorFormat=inherit  Unit=A  AffineConversion=off
  PS_i2b : nesl_utility/PS-Simulink Converter  PhysicalDomain=network_engine_domain  SubClassName=ps_output  LeftPortType=input  RightPortType=output  PseudoPeriodic=off  Frequencies=[]  VectorFormat=inherit  Unit=A  AffineConversion=off
  PS_i_mu : nesl_utility/PS-Simulink Converter  PhysicalDomain=network_engine_domain  SubClassName=ps_output  LeftPortType=input  RightPortType=output  PseudoPeriodic=off  Frequencies=[]  VectorFormat=inherit  Unit=A  AffineConversion=off
  PS_n : nesl_utility/PS-Simulink Converter  PhysicalDomain=network_engine_domain  SubClassName=ps_output  LeftPortType=input  RightPortType=output  PseudoPeriodic=off  Frequencies=[]  VectorFormat=inherit  Unit=rpm  AffineConversion=off
  PS_phi_el : Fcn  Expr=atan2(u(2),u(1))
  PS_psi_h : nesl_utility/PS-Simulink Converter  PhysicalDomain=network_engine_domain  SubClassName=ps_output  LeftPortType=input  RightPortType=output  PseudoPeriodic=off  Frequencies=[]  VectorFormat=inherit  Unit=Wb  AffineConversion=off
  PS_s : nesl_utility/PS-Simulink Converter  PhysicalDomain=network_engine_domain  SubClassName=ps_output  LeftPortType=input  RightPortType=output  PseudoPeriodic=off  Frequencies=[]  VectorFormat=inherit  Unit=1  AffineConversion=off
  PS_th_mech : nesl_utility/PS-Simulink Converter  PhysicalDomain=network_engine_domain  SubClassName=ps_output  LeftPortType=input  RightPortType=output  PseudoPeriodic=off  Frequencies=[]  VectorFormat=inherit  Unit=rad  AffineConversion=off
  PS_theta2 : Fcn  Expr=atan2(sin(atan2(u(2),u(1)) - p*u(3)), cos(atan2(u(2),u(1)) - p*u(3)))
  PS_u1 : nesl_utility/PS-Simulink Converter  PhysicalDomain=network_engine_domain  SubClassName=ps_output  LeftPortType=input  RightPortType=output  PseudoPeriodic=off  Frequencies=[]  VectorFormat=inherit  Unit=V  AffineConversion=off
  Stator : asmlib_lib/machine/Stator  R1=R1 Ohm  L1s=L1s H  iU_specify=off  iU_priority=None  iU=0 A  iU_nominal_specify=off  iU_nominal_value=1  iU_nominal_unit=A  iV_specify=off  iV_priority=None  iV=0 A  iV_nominal_specify=off  iV_nominal_value=1  iV_nominal_unit=A  iW_specify=off  iW_priority=None  iW=0 A  iW_nominal_specify=off  iW_nominal_value=1  iW_nominal_unit=A  i1ab_specify=off  i1ab_priority=None  i1ab=zeros(2, 1) A  i1ab_nominal_specify=off  i1ab_nominal_value=1  i1ab_nominal_unit=A  psih_specify=off  psih_priority=None  psih=zeros(2, 1) Wb  psih_nominal_specify=off  psih_nominal_value=1  psih_nominal_unit=Wb  psi1_specify=off  psi1_priority=High  psi1=zeros(2, 1) Wb  psi1_nominal_specify=off  psi1_nominal_value=1  psi1_nominal_unit=Wb  i0_specify=off  i0_priority=High  i0=0 A  i0_nominal_specify=off  i0_nominal_value=1  i0_nominal_unit=A
  mux_theta2 : Mux  Inputs=2
  a : PMIOPort  Side=Left
  b : PMIOPort  Port=2  Side=Left
  c : PMIOPort  Port=3  Side=Left
  R : PMIOPort  Port=4  Side=Right
  C : PMIOPort  Port=5  Side=Right
  Mess : Outport
  wires:
  PS_psi_h/1 -> PS_phi_el/1, mux_theta2/1, MeasBus/3  "psi_h"
  PS_th_mech/1 -> mux_theta2/2, MeasBus/11  "th_mech"
  mux_theta2/1 -> PS_theta2/1
  PS_i1/1 -> MeasBus/1  "i1"
  PS_u1/1 -> MeasBus/2  "u1"
  PS_phi_el/1 -> MeasBus/4  "phi_el"
  PS_Bhat/1 -> MeasBus/5  "Bhat"
  PS_i_mu/1 -> MeasBus/6  "i_mu"
  PS_i2b/1 -> MeasBus/7  "i2b"
  PS_M/1 -> MeasBus/8  "M"
  PS_n/1 -> MeasBus/9  "n"
  PS_Om/1 -> MeasBus/10  "Om"
  PS_theta2/1 -> MeasBus/12  "theta2"
  PS_s/1 -> MeasBus/13  "s"
  MeasBus/1 -> Mess/1
  connections:
  Klemmbrett/RConn1 -- Stator/LConn1
  Klemmbrett/RConn2 -- Stator/LConn2
  Klemmbrett/RConn3 -- Stator/LConn3
  Klemmbrett/RConn4 -- Stator/LConn4
  Klemmbrett/RConn5 -- Stator/LConn5
  Klemmbrett/RConn6 -- Stator/LConn6
  Käfigläufer/LConn1 -- Stator/RConn1 -- Luftspalt-Drehfeld/LConn1
  a/RConn1 -- Klemmbrett/LConn1
  b/RConn1 -- Klemmbrett/LConn2
  c/RConn1 -- Klemmbrett/LConn3
  R/RConn1 -- Käfigläufer/RConn1
  C/RConn1 -- Käfigläufer/RConn2
  Stator/RConn2 -- PS_i1/LConn1
  Stator/RConn3 -- PS_u1/LConn1
  Luftspalt-Drehfeld/RConn1 -- PS_psi_h/LConn1
  Luftspalt-Drehfeld/RConn2 -- PS_Bhat/LConn1
  Luftspalt-Drehfeld/RConn3 -- PS_i_mu/LConn1
  Käfigläufer/RConn3 -- PS_i2b/LConn1
  Käfigläufer/RConn4 -- PS_M/LConn1
  PS_n/LConn1 -- Käfigläufer/RConn5 -- PS_Om/LConn1
  Käfigläufer/RConn6 -- PS_th_mech/LConn1
  Käfigläufer/RConn7 -- PS_s/LConn1

== system asm_blocks_lib/Maschine/Klemmbrett ==
  terminal_box : asmlib_lib/machine/Terminal box  connection=connection  i_aU1_specify=off  i_aU1_priority=None  i_aU1=0 A  i_aU1_nominal_specify=off  i_aU1_nominal_value=1  i_aU1_nominal_unit=A  i_bV1_specify=off  i_bV1_priority=None  i_bV1=0 A  i_bV1_nominal_specify=off  i_bV1_nominal_value=1  i_bV1_nominal_unit=A  i_cW1_specify=off  i_cW1_priority=None  i_cW1=0 A  i_cW1_nominal_specify=off  i_cW1_nominal_value=1  i_cW1_nominal_unit=A  i_aW2_specify=off  i_aW2_priority=None  i_aW2=0 A  i_aW2_nominal_specify=off  i_aW2_nominal_value=1  i_aW2_nominal_unit=A  i_bU2_specify=off  i_bU2_priority=None  i_bU2=0 A  i_bU2_nominal_specify=off  i_bU2_nominal_value=1  i_bU2_nominal_unit=A  i_cV2_specify=off  i_cV2_priority=None  i_cV2=0 A  i_cV2_nominal_specify=off  i_cV2_nominal_value=1  i_cV2_nominal_unit=A  i_UV2_specify=off  i_UV2_priority=None  i_UV2=0 A  i_UV2_nominal_specify=off  i_UV2_nominal_value=1  i_UV2_nominal_unit=A  i_VW2_specify=off  i_VW2_priority=None  i_VW2=0 A  i_VW2_nominal_specify=off  i_VW2_nominal_value=1  i_VW2_nominal_unit=A
  a : PMIOPort  Side=Left
  b : PMIOPort  Port=2  Side=Left
  c : PMIOPort  Port=3  Side=Left
  U1 : PMIOPort  Port=4  Side=Right
  V1 : PMIOPort  Port=5  Side=Right
  W1 : PMIOPort  Port=6  Side=Right
  U2 : PMIOPort  Port=7  Side=Right
  V2 : PMIOPort  Port=8  Side=Right
  W2 : PMIOPort  Port=9  Side=Right
  connections:
  a/RConn1 -- terminal_box/LConn1
  b/RConn1 -- terminal_box/LConn2
  c/RConn1 -- terminal_box/LConn3
  U1/RConn1 -- terminal_box/RConn1
  V1/RConn1 -- terminal_box/RConn2
  W1/RConn1 -- terminal_box/RConn3
  U2/RConn1 -- terminal_box/RConn4
  V2/RConn1 -- terminal_box/RConn5
  W2/RConn1 -- terminal_box/RConn6

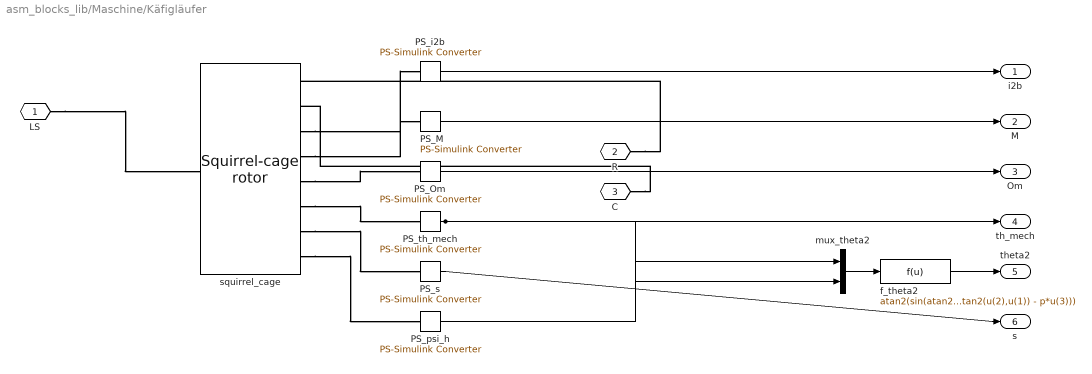
== system asm_blocks_lib/Maschine/Käfigläufer ==
  PS_M : nesl_utility/PS-Simulink Converter  PhysicalDomain=network_engine_domain  SubClassName=ps_output  LeftPortType=input  RightPortType=output  PseudoPeriodic=off  Frequencies=[]  VectorFormat=inherit  Unit=N*m  AffineConversion=off
  PS_Om : nesl_utility/PS-Simulink Converter  PhysicalDomain=network_engine_domain  SubClassName=ps_output  LeftPortType=input  RightPortType=output  PseudoPeriodic=off  Frequencies=[]  VectorFormat=inherit  Unit=rad/s  AffineConversion=off
  PS_i2b : nesl_utility/PS-Simulink Converter  PhysicalDomain=network_engine_domain  SubClassName=ps_output  LeftPortType=input  RightPortType=output  PseudoPeriodic=off  Frequencies=[]  VectorFormat=inherit  Unit=A  AffineConversion=off
  PS_psi_h : nesl_utility/PS-Simulink Converter  PhysicalDomain=network_engine_domain  SubClassName=ps_output  LeftPortType=input  RightPortType=output  PseudoPeriodic=off  Frequencies=[]  VectorFormat=inherit  Unit=Wb  AffineConversion=off
  PS_s : nesl_utility/PS-Simulink Converter  PhysicalDomain=network_engine_domain  SubClassName=ps_output  LeftPortType=input  RightPortType=output  PseudoPeriodic=off  Frequencies=[]  VectorFormat=inherit  Unit=1  AffineConversion=off
  PS_th_mech : nesl_utility/PS-Simulink Converter  PhysicalDomain=network_engine_domain  SubClassName=ps_output  LeftPortType=input  RightPortType=output  PseudoPeriodic=off  Frequencies=[]  VectorFormat=inherit  Unit=rad  AffineConversion=off
  f_theta2 : Fcn  Expr=atan2(sin(atan2(u(2),u(1)) - p*u(3)), cos(atan2(u(2),u(1)) - p*u(3)))
  mux_theta2 : Mux  Inputs=2
  squirrel_cage : asmlib_lib/machine/Squirrel-cage rotor  R2b=R2b Ohm  L2sb=L2sb H  p=p  f_N=f_N Hz  J_M=J_M kg*m^2  k_R=k_R N*m*s/rad  n0=n0 rpm  i2_specify=off  i2_priority=None  i2=zeros(2, 1) A  i2_nominal_specify=off  i2_nominal_value=1  i2_nominal_unit=A  psih_specify=off  psih_priority=None  psih=zeros(2, 1) Wb  psih_nominal_specify=off  psih_nominal_value=1  psih_nominal_unit=Wb  psi2_specify=off  psi2_priority=None  psi2=zeros(2, 1) Wb  psi2_nominal_specify=off  psi2_nominal_value=1  psi2_nominal_unit=Wb  psi2r_specify=off  psi2r_priority=High  psi2r=zeros(2, 1) Wb  psi2r_nominal_specify=off  psi2r_nominal_value=1  psi2r_nominal_unit=Wb  th_specify=off  th_priority=High  th=0 rad  th_nominal_specify=off  th_nominal_value=1  th_nominal_unit=rad  t_specify=off  t_priority=None  t=0 N*m  t_nominal_specify=off  t_nominal_value=1  t_nominal_unit=N*m  Mel_specify=off  Mel_priority=None  Mel=0 N*m  Mel_nominal_specify=off  Mel_nominal_value=1  Mel_nominal_unit=N*m
  LS : PMIOPort  Side=Left
  R : PMIOPort  Port=2  Side=Right
  C : PMIOPort  Port=3  Side=Right
  i2b : Outport
  M : Outport  Port=2
  Om : Outport  Port=3
  th_mech : Outport  Port=4
  theta2 : Outport  Port=5
  s : Outport  Port=6
  wires:
  PS_i2b/1 -> i2b/1
  PS_M/1 -> M/1
  PS_Om/1 -> Om/1
  PS_th_mech/1 -> th_mech/1, mux_theta2/2
  PS_psi_h/1 -> mux_theta2/1
  mux_theta2/1 -> f_theta2/1
  f_theta2/1 -> theta2/1
  PS_s/1 -> s/1
  connections:
  LS/RConn1 -- squirrel_cage/LConn1
  R/RConn1 -- squirrel_cage/RConn1
  C/RConn1 -- squirrel_cage/RConn2
  squirrel_cage/RConn3 -- PS_i2b/LConn1
  squirrel_cage/RConn4 -- PS_M/LConn1
  squirrel_cage/RConn5 -- PS_Om/LConn1
  squirrel_cage/RConn6 -- PS_th_mech/LConn1
  squirrel_cage/RConn7 -- PS_s/LConn1
  squirrel_cage/RConn8 -- PS_psi_h/LConn1

== system asm_blocks_lib/Maschine/Luftspalt-Drehfeld ==
  PS_Bhat : nesl_utility/PS-Simulink Converter  PhysicalDomain=network_engine_domain  SubClassName=ps_output  LeftPortType=input  RightPortType=output  PseudoPeriodic=off  Frequencies=[]  VectorFormat=inherit  Unit=T  AffineConversion=off
  PS_i_mu : nesl_utility/PS-Simulink Converter  PhysicalDomain=network_engine_domain  SubClassName=ps_output  LeftPortType=input  RightPortType=output  PseudoPeriodic=off  Frequencies=[]  VectorFormat=inherit  Unit=A  AffineConversion=off
  PS_psi_h : nesl_utility/PS-Simulink Converter  PhysicalDomain=network_engine_domain  SubClassName=ps_output  LeftPortType=input  RightPortType=output  PseudoPeriodic=off  Frequencies=[]  VectorFormat=inherit  Unit=Wb  AffineConversion=off
  airgap_field : asmlib_lib/machine/Air-gap field  Lh=Lh H  p=p  N1xi1=N1xi1  l=l m  r=r m  imu_specify=off  imu_priority=None  imu=zeros(2, 1) A  imu_nominal_specify=off  imu_nominal_value=1  imu_nominal_unit=A  psih_specify=off  psih_priority=None  psih=zeros(2, 1) Wb  psih_nominal_specify=off  psih_nominal_value=1  psih_nominal_unit=Wb
  f_phi_el : Fcn  Expr=atan2(u(2),u(1))
  LS : PMIOPort  Side=Left
  psi_h : Outport
  phi_el : Outport  Port=2
  Bhat : Outport  Port=3
  i_mu : Outport  Port=4
  wires:
  PS_psi_h/1 -> psi_h/1, f_phi_el/1
  f_phi_el/1 -> phi_el/1
  PS_Bhat/1 -> Bhat/1
  PS_i_mu/1 -> i_mu/1
  connections:
  LS/RConn1 -- airgap_field/LConn1
  airgap_field/RConn1 -- PS_psi_h/LConn1
  airgap_field/RConn2 -- PS_Bhat/LConn1
  airgap_field/RConn3 -- PS_i_mu/LConn1

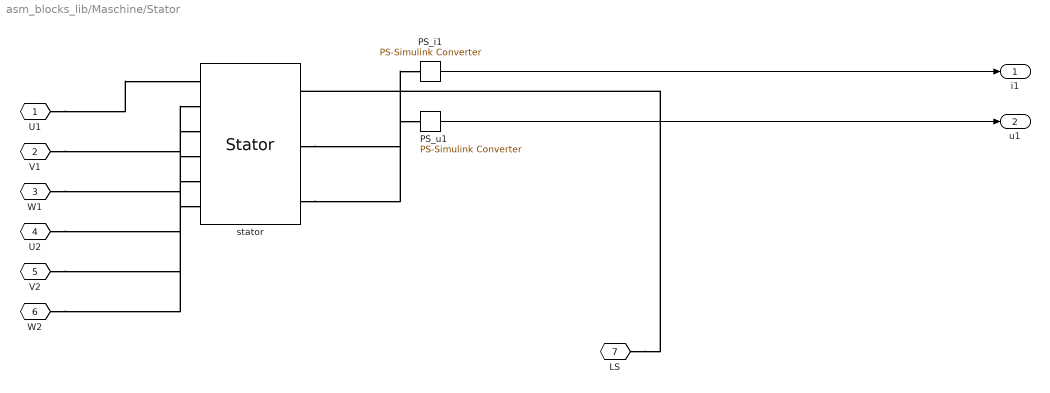
== system asm_blocks_lib/Maschine/Stator ==
  PS_i1 : nesl_utility/PS-Simulink Converter  PhysicalDomain=network_engine_domain  SubClassName=ps_output  LeftPortType=input  RightPortType=output  PseudoPeriodic=off  Frequencies=[]  VectorFormat=inherit  Unit=A  AffineConversion=off
  PS_u1 : nesl_utility/PS-Simulink Converter  PhysicalDomain=network_engine_domain  SubClassName=ps_output  LeftPortType=input  RightPortType=output  PseudoPeriodic=off  Frequencies=[]  VectorFormat=inherit  Unit=V  AffineConversion=off
  stator : asmlib_lib/machine/Stator  R1=R1 Ohm  L1s=L1s H  iU_specify=off  iU_priority=None  iU=0 A  iU_nominal_specify=off  iU_nominal_value=1  iU_nominal_unit=A  iV_specify=off  iV_priority=None  iV=0 A  iV_nominal_specify=off  iV_nominal_value=1  iV_nominal_unit=A  iW_specify=off  iW_priority=None  iW=0 A  iW_nominal_specify=off  iW_nominal_value=1  iW_nominal_unit=A  i1ab_specify=off  i1ab_priority=None  i1ab=zeros(2, 1) A  i1ab_nominal_specify=off  i1ab_nominal_value=1  i1ab_nominal_unit=A  psih_specify=off  psih_priority=None  psih=zeros(2, 1) Wb  psih_nominal_specify=off  psih_nominal_value=1  psih_nominal_unit=Wb  psi1_specify=off  psi1_priority=High  psi1=zeros(2, 1) Wb  psi1_nominal_specify=off  psi1_nominal_value=1  psi1_nominal_unit=Wb  i0_specify=off  i0_priority=High  i0=0 A  i0_nominal_specify=off  i0_nominal_value=1  i0_nominal_unit=A
  U1 : PMIOPort  Side=Left
  V1 : PMIOPort  Port=2  Side=Left
  W1 : PMIOPort  Port=3  Side=Left
  U2 : PMIOPort  Port=4  Side=Left
  V2 : PMIOPort  Port=5  Side=Left
  W2 : PMIOPort  Port=6  Side=Left
  LS : PMIOPort  Port=7  Side=Right
  i1 : Outport
  u1 : Outport  Port=2
  wires:
  PS_i1/1 -> i1/1
  PS_u1/1 -> u1/1
  connections:
  U1/RConn1 -- stator/LConn1
  V1/RConn1 -- stator/LConn2
  W1/RConn1 -- stator/LConn3
  U2/RConn1 -- stator/LConn4
  V2/RConn1 -- stator/LConn5
  W2/RConn1 -- stator/LConn6
  LS/RConn1 -- stator/RConn1
  stator/RConn2 -- PS_i1/LConn1
  stator/RConn3 -- PS_u1/LConn1

== system asm_blocks_lib/Mechanik/Last Kennlinie ==
  load_table : asmlib_lib/mechanics/Load from table  n_tab=n_tab rpm  M_tab=M_tab N*m  w_eps=0.1 rad/s  t_specify=off  t_priority=None  t=0 N*m  t_nominal_specify=off  t_nominal_value=1  t_nominal_unit=N*m  w_specify=off  w_priority=None  w=0 rad/s  w_nominal_specify=off  w_nominal_value=1  w_nominal_unit=rad/s
  R : PMIOPort  Side=Left
  C : PMIOPort  Port=2  Side=Right
  connections:
  R/RConn1 -- load_table/LConn1
  C/RConn1 -- load_table/RConn1

== system asm_blocks_lib/Mechanik/Last Lüfter ==
  load_fan : asmlib_lib/mechanics/Fan load  M_B=M_B N*m  n_B=n_B rpm  t_specify=off  t_priority=None  t=0 N*m  t_nominal_specify=off  t_nominal_value=1  t_nominal_unit=N*m  w_specify=off  w_priority=None  w=0 rad/s  w_nominal_specify=off  w_nominal_value=1  w_nominal_unit=rad/s
  R : PMIOPort  Side=Left
  C : PMIOPort  Port=2  Side=Right
  connections:
  R/RConn1 -- load_fan/LConn1
  C/RConn1 -- load_fan/RConn1

== system asm_blocks_lib/Mechanik/Last konstant ==
  load_constant : asmlib_lib/mechanics/Constant load  M_L0=M_L0 N*m  w_eps=0.1 rad/s  t_specify=off  t_priority=None  t=0 N*m  t_nominal_specify=off  t_nominal_value=1  t_nominal_unit=N*m  w_specify=off  w_priority=None  w=0 rad/s  w_nominal_specify=off  w_nominal_value=1  w_nominal_unit=rad/s
  R : PMIOPort  Side=Left
  C : PMIOPort  Port=2  Side=Right
  connections:
  R/RConn1 -- load_constant/LConn1
  C/RConn1 -- load_constant/RConn1

== system asm_blocks_lib/Mechanik/Laststoß ==
  load_step : asmlib_lib/mechanics/Load step  t_step=t_step s  dM_L=dM_L N*m  t_r=0.5e-3 s  w_eps=0.1 rad/s  t_specify=off  t_priority=None  t=0 N*m  t_nominal_specify=off  t_nominal_value=1  t_nominal_unit=N*m  w_specify=off  w_priority=None  w=0 rad/s  w_nominal_specify=off  w_nominal_value=1  w_nominal_unit=rad/s
  R : PMIOPort  Side=Left
  C : PMIOPort  Port=2  Side=Right
  connections:
  R/RConn1 -- load_step/LConn1
  C/RConn1 -- load_step/RConn1

== system asm_blocks_lib/Mechanik/Mechanischer Bezug ==
  mech_reference : fl_lib/Mechanical/Rotational Elements/Mechanical Rotational Reference
  C : PMIOPort  Side=Left
  connections:
  C/RConn1 -- mech_reference/LConn1

== system asm_blocks_lib/Mechanik/Reibung ==
  friction : asmlib_lib/mechanics/Friction  k_R=k_R N*m*s/rad  M_C=M_C N*m  w_eps=0.1 rad/s  t_specify=off  t_priority=None  t=0 N*m  t_nominal_specify=off  t_nominal_value=1  t_nominal_unit=N*m  w_specify=off  w_priority=None  w=0 rad/s  w_nominal_specify=off  w_nominal_value=1  w_nominal_unit=rad/s
  R : PMIOPort  Side=Left
  C : PMIOPort  Port=2  Side=Right
  connections:
  R/RConn1 -- friction/LConn1
  C/RConn1 -- friction/RConn1

== system asm_blocks_lib/Mechanik/Schwungmasse ==
  inertia : asmlib_lib/mechanics/Inertia  J=J kg*m^2  n0=n0 rpm  t_specify=off  t_priority=None  t=0 N*m  t_nominal_specify=off  t_nominal_value=1  t_nominal_unit=N*m
  R : PMIOPort  Side=Left
  connections:
  R/RConn1 -- inertia/LConn1
